simulink library "bushing_forces_lib"  (R2025a)
settings: Solver=VariableStepAuto  StartTime=0.0  StopTime=10.0  RelTol=1e-3
undefined symbols (not defined in the file): b1_radial_max, d_axial, d_axialX, d_axialY, d_axialZ, d_radial, d_tors, d_torsX, d_torsY, d_torsZ, f_axial_dam, f_axial_spr, f_axialX_dam, f_axialX_spr, f_axialY_dam, f_axialY_spr, f_axialZ_dam, f_axialZ_spr, f_radial_dam, f_radial_max, f_radial_spr, k1_radial_max, k_axial, k_axialX, k_axialY, k_axialZ, k_radial, k_tors, k_torsX, k_torsY, k_torsZ, Linear, m, m_spr, m_sprZ, m_torsY, m_torsZ, m_torX, q_spr, q_sprZ, Table, v_axial, v_axialX, v_axialY, v_axialZ, v_radial, w, w_torsY, w_torsZ, w_torX, x_axial, x_axialX, x_axialY, x_axialZ, x_radial, x_radial_max
libraries: nesl_utility x26, fl_lib x18, $bdroot x10
(part 1 of 2)
Description:
  | Copyright 2026 The MathWorks, Inc.
settings Model: Creator=smiller  LastModifiedBy=smiller
settings OptimizationCC: ReuseModelBlockBuffer=off
settings ModelReferenceCC: EnableRefExpFcnMdlSchedulingChecks=on
settings RTWCC: GPUComputeCapability=3.5

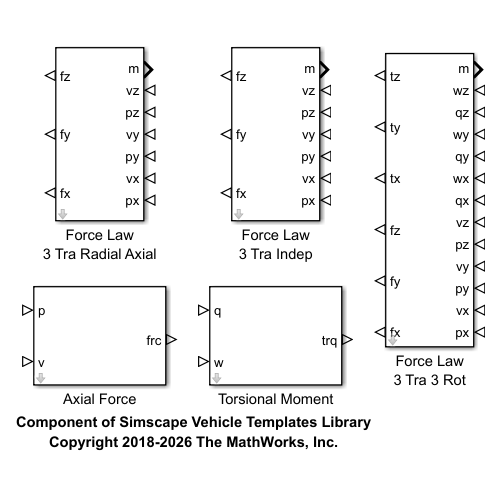
[thumbnail: Simulink's stored preview of the top-level diagram]
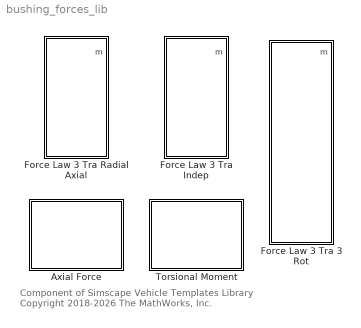
== system bushing_forces_lib ==
  note: Component of Simscape Vehicle Templates Library
      | Copyright 2018-2026 The MathWorks, Inc.
  Axial Force : Subsystem  mask(Axial Compliance){popup_force_law_spr=Linear, k_axial=k_axial, x_axial=x_axial, f_axial_spr=f_axial_spr, popup_force_law_dam=Linear, d_axial=d_axial, v_axial=v_axial, f_axial_dam=f_axial_dam}
      mask prompts: popup_force_law_spr "Spring Force Law"; k_axial "Spring Coefficient (N/mm)"; x_axial "Spring Displacement [min max] (mm)"; f_axial_spr "Spring Force [min max] (N)"; popup_force_law_dam "Damper Force Law"; d_axial "Damper Coefficient (N/(m/s))"; v_axial "Damper Velocity [min max] (m/s)"; f_axial_dam "Damper Force [min max] (N)"
      mask help: Models axial compliance of the bushing. Select force laws that model compliance as linear or nonlinear.
      mask TypeOptions popup_force_law_spr: Force Law Spring/popup_force_law
      mask Callback popup_force_law_spr:
      | maskObj = Simulink.Mask.get(gcb); % Get the mask object of the current block
      | kaxi_h  = maskObj.getParameter('k_axial'); % Get the parameter to hide
      | 
      | xaxi_h  = maskObj.getParameter('x_axial'); % Get the parameter to hide
      | fSaxi_h  = maskObj.getParameter('f_axial_spr'); % Get the parameter to hide
      | 
      | % Check the value of ControlParam
      | controlParamValue = get_param(gcb, 'popup_force_law_spr');
      | 
      | kaxi_h.Visible  = 'off';
      | xaxi_h.Visible  = 'off';
      | fSaxi_h.Visible  = 'off';
      | 
      | if strcmp(controlParamValue, 'Linear')
      |     kaxi_h.Visible  = 'on';
      | else
      |     xaxi_h.Visible  = 'on';
      |     fSaxi_h.Visible  = 'on';
      | end
      mask TypeOptions k_axial: Force Law Spring/k_axial
      mask TypeOptions x_axial: Force Law Spring/x_axial
      mask TypeOptions f_axial_spr: Force Law Spring/f_axial
      mask TypeOptions popup_force_law_dam: Force Law Damping/popup_force_law
      mask Callback popup_force_law_dam:
      | maskObj = Simulink.Mask.get(gcb); % Get the mask object of the current block
      | daxi_h  = maskObj.getParameter('d_axial'); % Get the parameter to hide
      | 
      | vaxi_h  = maskObj.getParameter('v_axial'); % Get the parameter to hide
      | fDaxi_h  = maskObj.getParameter('f_axial_dam'); % Get the parameter to hide
      | 
      | % Check the value of ControlParam
      | controlParamValue = get_param(gcb, 'popup_force_law_dam');
      | 
      | daxi_h.Visible  = 'off';
      | vaxi_h.Visible  = 'off';
      | fDaxi_h.Visible  = 'off';
      | 
      | if strcmp(controlParamValue, 'Linear')
      |     daxi_h.Visible  = 'on';
      | else
      |     vaxi_h.Visible  = 'on';
      |     fDaxi_h.Visible  = 'on';
      | end
      mask TypeOptions d_axial: Force Law Damping/d_axial
      mask TypeOptions v_axial: Force Law Damping/v_axial
      mask TypeOptions f_axial_dam: Force Law Damping/f_axial
      mask DialogControl cont_radial Prompt: Radial
  Force Law 3 Tra 3 Rot : Subsystem  mask(Bushing Compliance){popup_force_law_spr_axiX=Linear, k_axialX=k_axialX, x_axialX=x_axialX, f_axialX_spr=f_axialX_spr, popup_force_law_dam_axiX=Linear, d_axialX=d_axialX, v_axialX=v_axialX, f_axialX_dam=f_axialX_dam, popup_force_law_spr_axiY=Linear, k_axialY=k_axialY, x_axialY=x_axialY, f_axialY_spr=f_axialY_spr, popup_force_law_dam_axiY=Linear, d_axialY=d_axialY, v_axialY=v_axialY, f_axialY_dam=f_axialY_dam, popup_force_law_spr_axiZ=Linear, k_axialZ=k_axialZ, x_axialZ=x_axialZ, f_axialZ_spr=f_axialZ_spr, popup_force_law_dam_axiZ=Linear, d_axialZ=d_axialZ, f_axialZ_dam=f_axialZ_dam, v_axialZ=v_axialZ, popup_force_law_spr_torX=Linear, k_torsX=k_torsX, q_sprX=q_spr, m_sprX=m_spr, popup_force_law_dam_torX=Linear, d_torsX=d_torsX, w_torsX=w_torX, m_torsX=m_torX, popup_force_law_spr_torY=Table, k_torsY=k_torsY, q_sprY=q_spr, m_sprY=m_spr, popup_force_law_dam_torY=Table, d_torsY=d_torsY, w_torsY=w_torsY, m_torsY=m_torsY, popup_force_law_spr_torZ=Linear, k_torsZ=k_torsZ, q_sprZ=q_sprZ, m_sprZ=m_sprZ, popup_force_law_dam_torZ=Linear, d_torsZ=d_torsZ, w_torsZ=w_torsZ, m_torsZ=m_torsZ}
      mask prompts: popup_force_law_spr_axiX "Spring Force Law"; k_axialX "Spring Coefficient (N/mm)"; x_axialX "Spring Displacement [min max] (mm)"; f_axialX_spr "Spring Force [min max] (N)"; popup_force_law_dam_axiX "Damper Force Law"; d_axialX "Damper Coefficient (N/(m/s))"; v_axialX "Damper Velocity [min max] (m/s)"; f_axialX_dam "Damper Force [min max] (N)"; popup_force_law_spr_axiY "Spring Force Law"; k_axialY "Spring Coefficient (N/mm)"; x_axialY "Spring Displacement [min max] (mm)"; f_axialY_spr "Spring Force [min max] (N)"; popup_force_law_dam_axiY "Damper Force Law"; d_axialY "Damper Coefficient (N/(m/s))"; v_axialY "Damper Velocity [min max] (m/s)"; f_axialY_dam "Damper Force [min max] (N)"; popup_force_law_spr_axiZ "Spring Force Law"; k_axialZ "Spring Coefficient (N/mm)"; x_axialZ "Spring Displacement [min max] (mm)"; f_axialZ_spr "Spring Force [min max] (N)"; popup_force_law_dam_axiZ "Damper Force Law"; d_axialZ "Damper Coefficient (N/(m/s))"; f_axialZ_dam "Damper Force [min max] (N)"; v_axialZ "Damper Velocity [min max] (m/s)"; popup_force_law_spr_torX "Spring Force Law"; k_torsX "Spring Coefficient  (N*m/deg)"; q_sprX "Spring Displacement [min max] (deg)"; m_sprX "Spring Torque [min max] (N*m)"; popup_force_law_dam_torX "Damper Force Law"; d_torsX "Damper Coefficient (N*m/(deg/s))"; w_torsX "Damper Velocity [min max] (deg/s)"; m_torsX "Damper Torque [min max] (N*m)"; popup_force_law_spr_torY "Spring Force Law"; k_torsY "Spring Coefficient (N*m/deg)"; q_sprY "Spring Displacement [min max] (deg)"; m_sprY "Spring Torque [min max] (N*m)"; popup_force_law_dam_torY "Damper Force Law"; d_torsY "Damper Coefficient (N*m/(deg/s))"; w_torsY "Damper Velocity [min max] (deg/s)"; m_torsY "Damper Torque [min max] (N*m)"; popup_force_law_spr_torZ "Spring Force Law"; k_torsZ "Spring Coefficient (N*m/deg)"; q_sprZ "Spring Displacement [min max] (deg)"; m_sprZ "Spring Torque [min max] (N*m)"; popup_force_law_dam_torZ "Damper Force Law"; d_torsZ "Damper Coefficient (N*m/(deg/s))"; w_torsZ "Damper Velocity [min max] (deg/s)"; m_torsZ "Damper Torque [min max] (N*m)"
      mask help: Models radial and axial compliance of the bushing. Select force laws that model compliance as linear or nonlinear.
      mask TypeOptions popup_force_law_spr_axiX: Force X/popup_force_law_spr
      mask Callback popup_force_law_spr_axiX:
      | maskObj = Simulink.Mask.get(gcb); % Get the mask object of the current block
      | kaxiX_h  = maskObj.getParameter('k_axialX'); % Get the parameter to hide
      | 
      | xaxiX_h  = maskObj.getParameter('x_axialX'); % Get the parameter to hide
      | fSaxiX_h  = maskObj.getParameter('f_axialX_spr'); % Get the parameter to hide
      | 
      | % Check the value of ControlParam
      | controlParamValue = get_param(gcb, 'popup_force_law_spr_axiX');
      | 
      | kaxiX_h.Visible  = 'off';
      | xaxiX_h.Visible  = 'off';
      | fSaxiX_h.Visible  = 'off';
      | 
      | if strcmp(controlParamValue, 'Linear')
      |     kaxiX_h.Visible  = 'on';
      | elseif strcmp(controlParamValue, 'Table')
      |     xaxiX_h.Visible  = 'on';
      |     fSaxiX_h.Visible  = 'on';
      | end
      mask TypeOptions k_axialX: Force X/k_axial
      mask TypeOptions x_axialX: Force X/x_axial
      mask TypeOptions f_axialX_spr: Force X/f_axial_spr
      mask TypeOptions popup_force_law_dam_axiX: Force X/popup_force_law_dam
      mask Callback popup_force_law_dam_axiX:
      | maskObj = Simulink.Mask.get(gcb); % Get the mask object of the current block
      | daxiX_h  = maskObj.getParameter('d_axialX'); % Get the parameter to hide
      | 
      | vaxiX_h  = maskObj.getParameter('v_axialX'); % Get the parameter to hide
      | fDaxiX_h  = maskObj.getParameter('f_axialX_dam'); % Get the parameter to hide
      | 
      | % Check the value of ControlParam
      | controlParamValue = get_param(gcb, 'popup_force_law_dam_axiX');
      | 
      | daxiX_h.Visible  = 'off';
      | vaxiX_h.Visible  = 'off';
      | fDaxiX_h.Visible  = 'off';
      | 
      | if strcmp(controlParamValue, 'Linear')
      |     daxiX_h.Visible  = 'on';
      | else
      |     vaxiX_h.Visible  = 'on';
      |     fDaxiX_h.Visible  = 'on';
      | end
      mask TypeOptions d_axialX: Force X/d_axial
      mask TypeOptions v_axialX: Force X/v_axial
      mask TypeOptions f_axialX_dam: Force X/f_axial_dam
      mask TypeOptions popup_force_law_spr_axiY: Force Y/popup_force_law_spr
      mask Callback popup_force_law_spr_axiY:
      | maskObj = Simulink.Mask.get(gcb); % Get the mask object of the current block
      | kaxiY_h  = maskObj.getParameter('k_axialY'); % Get the parameter to hide
      | 
      | xaxiY_h  = maskObj.getParameter('x_axialY'); % Get the parameter to hide
      | fSaxiY_h  = maskObj.getParameter('f_axialY_spr'); % Get the parameter to hide
      | 
      | % Check the value of ControlParam
      | controlParamValue = get_param(gcb, 'popup_force_law_spr_axiY');
      | 
      | kaxiY_h.Visible  = 'off';
      | xaxiY_h.Visible  = 'off';
      | fSaxiY_h.Visible  = 'off';
      | 
      | if strcmp(controlParamValue, 'Linear')
      |     kaxiY_h.Visible  = 'on';
      | elseif strcmp(controlParamValue, 'Table')
      |     xaxiY_h.Visible  = 'on';
      |     fSaxiY_h.Visible  = 'on';
      | end
      mask TypeOptions k_axialY: Force Y/k_axial
      mask TypeOptions x_axialY: Force Y/x_axial
      mask TypeOptions f_axialY_spr: Force Y/f_axial_spr
      mask TypeOptions popup_force_law_dam_axiY: Force Y/popup_force_law_dam
      mask Callback popup_force_law_dam_axiY:
      | maskObj = Simulink.Mask.get(gcb); % Get the mask object of the current block
      | daxiY_h  = maskObj.getParameter('d_axialY'); % Get the parameter to hide
      | 
      | vaxiY_h  = maskObj.getParameter('v_axialY'); % Get the parameter to hide
      | fDaxiY_h  = maskObj.getParameter('f_axialY_dam'); % Get the parameter to hide
      | 
      | % Check the value of ControlParam
      | controlParamValue = get_param(gcb, 'popup_force_law_dam_axiY');
      | 
      | daxiY_h.Visible  = 'off';
      | vaxiY_h.Visible  = 'off';
      | fDaxiY_h.Visible  = 'off';
      | 
      | if strcmp(controlParamValue, 'Linear')
      |     daxiY_h.Visible  = 'on';
      | else
      |     vaxiY_h.Visible  = 'on';
      |     fDaxiY_h.Visible  = 'on';
      | end
      mask TypeOptions d_axialY: Force Y/d_axial
      mask TypeOptions v_axialY: Force Y/v_axial
      mask TypeOptions f_axialY_dam: Force Y/f_axial_dam
      mask TypeOptions popup_force_law_spr_axiZ: Force Z/popup_force_law_spr
      mask Callback popup_force_law_spr_axiZ:
      | maskObj = Simulink.Mask.get(gcb); % Get the mask object of the current block
      | kaxiZ_h  = maskObj.getParameter('k_axialZ'); % Get the parameter to hide
      | 
      | xaxiZ_h  = maskObj.getParameter('x_axialZ'); % Get the parameter to hide
      | fSaxiZ_h  = maskObj.getParameter('f_axialZ_spr'); % Get the parameter to hide
      | 
      | % Check the value of ControlParam
      | controlParamValue = get_param(gcb, 'popup_force_law_spr_axiZ');
      | 
      | kaxiZ_h.Visible  = 'off';
      | xaxiZ_h.Visible  = 'off';
      | fSaxiZ_h.Visible  = 'off';
      | 
      | if strcmp(controlParamValue, 'Linear')
      |     kaxiZ_h.Visible  = 'on';
      | elseif strcmp(controlParamValue, 'Table')
      |     xaxiZ_h.Visible  = 'on';
      |     fSaxiZ_h.Visible  = 'on';
      | end
      mask TypeOptions k_axialZ: Force Z/k_axial
      mask TypeOptions x_axialZ: Force Z/x_axial
      mask TypeOptions f_axialZ_spr: Force Z/f_axial_spr
      mask TypeOptions popup_force_law_dam_axiZ: Force Z/popup_force_law_dam
      mask Callback popup_force_law_dam_axiZ:
      | maskObj = Simulink.Mask.get(gcb); % Get the mask object of the current block
      | daxiZ_h  = maskObj.getParameter('d_axialZ'); % Get the parameter to hide
      | 
      | vaxiZ_h  = maskObj.getParameter('v_axialZ'); % Get the parameter to hide
      | fDaxiZ_h  = maskObj.getParameter('f_axialZ_dam'); % Get the parameter to hide
      | 
      | % Check the value of ControlParam
      | controlParamValue = get_param(gcb, 'popup_force_law_dam_axiZ');
      | 
      | daxiZ_h.Visible  = 'off';
      | vaxiZ_h.Visible  = 'off';
      | fDaxiZ_h.Visible  = 'off';
      | 
      | if strcmp(controlParamValue, 'Linear')
      |     daxiZ_h.Visible  = 'on';
      | else
      |     vaxiZ_h.Visible  = 'on';
      |     fDaxiZ_h.Visible  = 'on';
      | end
      mask TypeOptions d_axialZ: Force Z/d_axial
      mask TypeOptions f_axialZ_dam: Force Z/f_axial_dam
      mask TypeOptions v_axialZ: Force Z/v_axial
      mask TypeOptions popup_force_law_spr_torX: Torque X/popup_force_law_spr
      mask Callback popup_force_law_spr_torX:
      | maskObj = Simulink.Mask.get(gcb); % Get the mask object of the current block
      | ktorX_h  = maskObj.getParameter('k_torsX'); % Get the parameter to hide
      | 
      | qsprX_h  = maskObj.getParameter('q_sprX'); % Get the parameter to hide
      | msprX_h  = maskObj.getParameter('m_sprX'); % Get the parameter to hide
      | 
      | % Check the value of ControlParam
      | controlParamValue = get_param(gcb, 'popup_force_law_spr_torX');
      | 
      | ktorX_h.Visible  = 'off';
      | qsprX_h.Visible  = 'off';
      | msprX_h.Visible  = 'off';
      | 
      | if strcmp(controlParamValue, 'Linear')
      |     ktorX_h.Visible  = 'on';
      | elseif strcmp(controlParamValue, 'Table')
      |     qsprX_h.Visible  = 'on';
      |     msprX_h.Visible  = 'on';
      | end
      mask TypeOptions k_torsX: Torque X/k_tors
      mask TypeOptions q_sprX: Torque X/q_spr
      mask TypeOptions m_sprX: Torque X/m_spr
      mask TypeOptions popup_force_law_dam_torX: Torque X/popup_force_law_dam
      mask Callback popup_force_law_dam_torX:
      | maskObj = Simulink.Mask.get(gcb); % Get the mask object of the current block
      | dtorX_h  = maskObj.getParameter('d_torsX'); % Get the parameter to hide
      | 
      | wtorX_h  = maskObj.getParameter('w_torsX'); % Get the parameter to hide
      | mtorX_h  = maskObj.getParameter('m_torsX'); % Get the parameter to hide
      | 
      | % Check the value of ControlParam
      | controlParamValue = get_param(gcb, 'popup_force_law_dam_torX');
      | 
      | dtorX_h.Visible  = 'off';
      | wtorX_h.Visible  = 'off';
      | mtorX_h.Visible  = 'off';
      | 
      | if strcmp(controlParamValue, 'Linear')
      |     dtorX_h.Visible  = 'on';
      | else
      |     wtorX_h.Visible  = 'on';
      |     mtorX_h.Visible  = 'on';
      | end
      mask TypeOptions d_torsX: Torque X/d_tors
      mask TypeOptions w_torsX: Torque X/w
      mask TypeOptions m_torsX: Torque X/m
      mask TypeOptions popup_force_law_spr_torY: Torque Y/popup_force_law_spr
      mask Callback popup_force_law_spr_torY:
      | maskObj = Simulink.Mask.get(gcb); % Get the mask object of the current block
      | ktorY_h  = maskObj.getParameter('k_torsY'); % Get the parameter to hide
      | 
      | qsprY_h  = maskObj.getParameter('q_sprY'); % Get the parameter to hide
      | msprY_h  = maskObj.getParameter('m_sprY'); % Get the parameter to hide
      | 
      | % Check the value of ControlParam
      | controlParamValue = get_param(gcb, 'popup_force_law_spr_torY');
      | 
      | ktorY_h.Visible  = 'off';
      | qsprY_h.Visible  = 'off';
      | msprY_h.Visible  = 'off';
      | 
      | if strcmp(controlParamValue, 'Linear')
      |     ktorY_h.Visible  = 'on';
      | elseif strcmp(controlParamValue, 'Table')
      |     qsprY_h.Visible  = 'on';
      |     msprY_h.Visible  = 'on';
      | end
      mask TypeOptions k_torsY: Torque Y/k_tors
      mask TypeOptions q_sprY: Torque Y/q_spr
      mask TypeOptions m_sprY: Torque Y/m_spr
      mask TypeOptions popup_force_law_dam_torY: Torque Y/popup_force_law_dam
      mask Callback popup_force_law_dam_torY:
      | maskObj = Simulink.Mask.get(gcb); % Get the mask object of the current block
      | dtorY_h  = maskObj.getParameter('d_torsY'); % Get the parameter to hide
      | 
      | wtorY_h  = maskObj.getParameter('w_torsY'); % Get the parameter to hide
      | mtorY_h  = maskObj.getParameter('m_torsY'); % Get the parameter to hide
      | 
      | % Check the value of ControlParam
      | controlParamValue = get_param(gcb, 'popup_force_law_dam_torY');
      | 
      | dtorY_h.Visible  = 'off';
      | wtorY_h.Visible  = 'off';
      | mtorY_h.Visible  = 'off';
      | 
      | if strcmp(controlParamValue, 'Linear')
      |     dtorY_h.Visible  = 'on';
      | else
      |     wtorY_h.Visible  = 'on';
      |     mtorY_h.Visible  = 'on';
      | end
      mask TypeOptions d_torsY: Torque Y/d_tors
      mask TypeOptions w_torsY: Torque Y/w
      mask TypeOptions m_torsY: Torque Y/m
      mask TypeOptions popup_force_law_spr_torZ: Torque Z/popup_force_law_spr
      mask Callback popup_force_law_spr_torZ:
      | maskObj = Simulink.Mask.get(gcb); % Get the mask object of the current block
      | ktorZ_h  = maskObj.getParameter('k_torsZ'); % Get the parameter to hide
      | 
      | qsprZ_h  = maskObj.getParameter('q_sprZ'); % Get the parameter to hide
      | msprZ_h  = maskObj.getParameter('m_sprZ'); % Get the parameter to hide
      | 
      | % Check the value of ControlParam
      | controlParamValue = get_param(gcb, 'popup_force_law_spr_torZ');
      | 
      | ktorZ_h.Visible  = 'off';
      | qsprZ_h.Visible  = 'off';
      | msprZ_h.Visible  = 'off';
      | 
      | if strcmp(controlParamValue, 'Linear')
      |     ktorZ_h.Visible  = 'on';
      | elseif strcmp(controlParamValue, 'Table')
      |     qsprZ_h.Visible  = 'on';
      |     msprZ_h.Visible  = 'on';
      | end
      mask TypeOptions k_torsZ: Torque Z/k_tors
      mask TypeOptions q_sprZ: Torque Z/q_spr
      mask TypeOptions m_sprZ: Torque Z/m_spr
      mask TypeOptions popup_force_law_dam_torZ: Torque Z/popup_force_law_dam
      mask Callback popup_force_law_dam_torZ:
      | maskObj = Simulink.Mask.get(gcb); % Get the mask object of the current block
      | dtorZ_h  = maskObj.getParameter('d_torsZ'); % Get the parameter to hide
      | 
      | wtorZ_h  = maskObj.getParameter('w_torsZ'); % Get the parameter to hide
      | mtorZ_h  = maskObj.getParameter('m_torsZ'); % Get the parameter to hide
      | 
      | % Check the value of ControlParam
      | controlParamValue = get_param(gcb, 'popup_force_law_dam_torZ');
      | 
      | dtorZ_h.Visible  = 'off';
      | wtorZ_h.Visible  = 'off';
      | mtorZ_h.Visible  = 'off';
      | 
      | if strcmp(controlParamValue, 'Linear')
      |     dtorZ_h.Visible  = 'on';
      | else
      |     wtorZ_h.Visible  = 'on';
      |     mtorZ_h.Visible  = 'on';
      | end
      mask TypeOptions d_torsZ: Torque Z/d_tors
      mask TypeOptions w_torsZ: Torque Z/w
      mask TypeOptions m_torsZ: Torque Z/m
      mask DialogControl cont_axialX Prompt: Axial (local x)
      mask DialogControl cont_axialY Prompt: Axial (local y)
      mask DialogControl cont_axialZ Prompt: Axial (local z)
      mask DialogControl cont_torsX Prompt: Torsional (local x)
      mask DialogControl cont_torsY Prompt: Torsional (local y)
      mask DialogControl cont_torsZ Prompt: Torsional (local z)
  Force Law 3 Tra Indep : Subsystem  mask(Bushing Compliance){popup_force_law_spr_axiX=Linear, k_axialX=k_axialX, x_axialX=x_axialX, f_axialX_spr=f_axialX_spr, popup_force_law_dam_axiX=Linear, d_axialX=d_axialX, v_axialX=v_axialX, f_axialX_dam=f_axialX_dam, popup_force_law_spr_axiY=Linear, k_axialY=k_axialY, x_axialY=x_axialY, f_axialY_spr=f_axialY_spr, popup_force_law_dam_axiY=Linear, d_axialY=d_axialY, v_axialY=v_axialY, f_axialY_dam=f_axialY_dam, popup_force_law_spr_axiZ=Linear, k_axialZ=k_axialZ, x_axialZ=x_axialZ, f_axialZ_spr=f_axialZ_spr, popup_force_law_dam_axiZ=Linear, d_axialZ=d_axialZ, f_axialZ_dam=f_axialZ_dam, v_axialZ=v_axialZ}
      mask prompts: popup_force_law_spr_axiX "Spring Force Law"; k_axialX "Spring Coefficient (N/mm)"; x_axialX "Spring Displacement [min max] (mm)"; f_axialX_spr "Spring Force [min max] (N)"; popup_force_law_dam_axiX "Damper Force Law"; d_axialX "Damper Coefficient (N/(m/s))"; v_axialX "Damper Velocity [min max] (m/s)"; f_axialX_dam "Damper Force [min max] (N)"; popup_force_law_spr_axiY "Spring Force Law"; k_axialY "Spring Coefficient (N/mm)"; x_axialY "Spring Displacement [min max] (mm)"; f_axialY_spr "Spring Force [min max] (N)"; popup_force_law_dam_axiY "Damper Force Law"; d_axialY "Damper Coefficient (N/(m/s))"; v_axialY "Damper Velocity [min max] (m/s)"; f_axialY_dam "Damper Force [min max] (N)"; popup_force_law_spr_axiZ "Spring Force Law"; k_axialZ "Spring Coefficient (N/mm)"; x_axialZ "Spring Displacement [min max] (mm)"; f_axialZ_spr "Spring Force [min max] (N)"; popup_force_law_dam_axiZ "Damper Force Law"; d_axialZ "Damper Coefficient (N/(m/s))"; f_axialZ_dam "Damper Force [min max] (N)"; v_axialZ "Damper Velocity [min max] (m/s)"
      mask help: Models radial and axial compliance of the bushing. Select force laws that model compliance as linear or nonlinear.
      mask TypeOptions popup_force_law_spr_axiX: Force X/popup_force_law_spr
      mask Callback popup_force_law_spr_axiX:
      | maskObj = Simulink.Mask.get(gcb); % Get the mask object of the current block
      | kaxiX_h  = maskObj.getParameter('k_axialX'); % Get the parameter to hide
      | 
      | xaxiX_h  = maskObj.getParameter('x_axialX'); % Get the parameter to hide
      | fSaxiX_h  = maskObj.getParameter('f_axialX_spr'); % Get the parameter to hide
      | 
      | % Check the value of ControlParam
      | controlParamValue = get_param(gcb, 'popup_force_law_spr_axiX');
      | 
      | kaxiX_h.Visible  = 'off';
      | xaxiX_h.Visible  = 'off';
      | fSaxiX_h.Visible  = 'off';
      | 
      | if strcmp(controlParamValue, 'Linear')
      |     kaxiX_h.Visible  = 'on';
      | elseif strcmp(controlParamValue, 'Table')
      |     xaxiX_h.Visible  = 'on';
      |     fSaxiX_h.Visible  = 'on';
      | end
      mask TypeOptions k_axialX: Force X/k_axial
      mask TypeOptions x_axialX: Force X/x_axial
      mask TypeOptions f_axialX_spr: Force X/f_axial_spr
      mask TypeOptions popup_force_law_dam_axiX: Force X/popup_force_law_dam
      mask Callback popup_force_law_dam_axiX:
      | maskObj = Simulink.Mask.get(gcb); % Get the mask object of the current block
      | daxiX_h  = maskObj.getParameter('d_axialX'); % Get the parameter to hide
      | 
      | vaxiX_h  = maskObj.getParameter('v_axialX'); % Get the parameter to hide
      | fDaxiX_h  = maskObj.getParameter('f_axialX_dam'); % Get the parameter to hide
      | 
      | % Check the value of ControlParam
      | controlParamValue = get_param(gcb, 'popup_force_law_dam_axiX');
      | 
      | daxiX_h.Visible  = 'off';
      | vaxiX_h.Visible  = 'off';
      | fDaxiX_h.Visible  = 'off';
      | 
      | if strcmp(controlParamValue, 'Linear')
      |     daxiX_h.Visible  = 'on';
      | else
      |     vaxiX_h.Visible  = 'on';
      |     fDaxiX_h.Visible  = 'on';
      | end
      mask TypeOptions d_axialX: Force X/d_axial
      mask TypeOptions v_axialX: Force X/v_axial
      mask TypeOptions f_axialX_dam: Force X/f_axial_dam
      mask TypeOptions popup_force_law_spr_axiY: Force Y/popup_force_law_spr
      mask Callback popup_force_law_spr_axiY:
      | maskObj = Simulink.Mask.get(gcb); % Get the mask object of the current block
      | kaxiY_h  = maskObj.getParameter('k_axialY'); % Get the parameter to hide
      | 
      | xaxiY_h  = maskObj.getParameter('x_axialY'); % Get the parameter to hide
      | fSaxiY_h  = maskObj.getParameter('f_axialY_spr'); % Get the parameter to hide
      | 
      | % Check the value of ControlParam
      | controlParamValue = get_param(gcb, 'popup_force_law_spr_axiY');
      | 
      | kaxiY_h.Visible  = 'off';
      | xaxiY_h.Visible  = 'off';
      | fSaxiY_h.Visible  = 'off';
      | 
      | if strcmp(controlParamValue, 'Linear')
      |     kaxiY_h.Visible  = 'on';
      | elseif strcmp(controlParamValue, 'Table')
      |     xaxiY_h.Visible  = 'on';
      |     fSaxiY_h.Visible  = 'on';
      | end
      mask TypeOptions k_axialY: Force Y/k_axial
      mask TypeOptions x_axialY: Force Y/x_axial
      mask TypeOptions f_axialY_spr: Force Y/f_axial_spr
      mask TypeOptions popup_force_law_dam_axiY: Force Y/popup_force_law_dam
      mask Callback popup_force_law_dam_axiY:
      | maskObj = Simulink.Mask.get(gcb); % Get the mask object of the current block
      | daxiY_h  = maskObj.getParameter('d_axialY'); % Get the parameter to hide
      | 
      | vaxiY_h  = maskObj.getParameter('v_axialY'); % Get the parameter to hide
      | fDaxiY_h  = maskObj.getParameter('f_axialY_dam'); % Get the parameter to hide
      | 
      | % Check the value of ControlParam
      | controlParamValue = get_param(gcb, 'popup_force_law_dam_axiY');
      | 
      | daxiY_h.Visible  = 'off';
      | vaxiY_h.Visible  = 'off';
      | fDaxiY_h.Visible  = 'off';
      | 
      | if strcmp(controlParamValue, 'Linear')
      |     daxiY_h.Visible  = 'on';
      | else
      |     vaxiY_h.Visible  = 'on';
      |     fDaxiY_h.Visible  = 'on';
      | end
      mask TypeOptions d_axialY: Force Y/d_axial
      mask TypeOptions v_axialY: Force Y/v_axial
      mask TypeOptions f_axialY_dam: Force Y/f_axial_dam
      mask TypeOptions popup_force_law_spr_axiZ: Force Z/popup_force_law_spr
      mask Callback popup_force_law_spr_axiZ:
      | maskObj = Simulink.Mask.get(gcb); % Get the mask object of the current block
      | kaxiZ_h  = maskObj.getParameter('k_axialZ'); % Get the parameter to hide
      | 
      | xaxiZ_h  = maskObj.getParameter('x_axialZ'); % Get the parameter to hide
      | fSaxiZ_h  = maskObj.getParameter('f_axialZ_spr'); % Get the parameter to hide
      | 
      | % Check the value of ControlParam
      | controlParamValue = get_param(gcb, 'popup_force_law_spr_axiZ');
      | 
      | kaxiZ_h.Visible  = 'off';
      | xaxiZ_h.Visible  = 'off';
      | fSaxiZ_h.Visible  = 'off';
      | 
      | if strcmp(controlParamValue, 'Linear')
      |     kaxiZ_h.Visible  = 'on';
      | elseif strcmp(controlParamValue, 'Table')
      |     xaxiZ_h.Visible  = 'on';
      |     fSaxiZ_h.Visible  = 'on';
      | end
      mask TypeOptions k_axialZ: Force Z/k_axial
      mask TypeOptions x_axialZ: Force Z/x_axial
      mask TypeOptions f_axialZ_spr: Force Z/f_axial_spr
      mask TypeOptions popup_force_law_dam_axiZ: Force Z/popup_force_law_dam
      mask Callback popup_force_law_dam_axiZ:
      | maskObj = Simulink.Mask.get(gcb); % Get the mask object of the current block
      | daxiZ_h  = maskObj.getParameter('d_axialZ'); % Get the parameter to hide
      | 
      | vaxiZ_h  = maskObj.getParameter('v_axialZ'); % Get the parameter to hide
      | fDaxiZ_h  = maskObj.getParameter('f_axialZ_dam'); % Get the parameter to hide
      | 
      | % Check the value of ControlParam
      | controlParamValue = get_param(gcb, 'popup_force_law_dam_axiZ');
      | 
      | daxiZ_h.Visible  = 'off';
      | vaxiZ_h.Visible  = 'off';
      | fDaxiZ_h.Visible  = 'off';
      | 
      | if strcmp(controlParamValue, 'Linear')
      |     daxiZ_h.Visible  = 'on';
      | else
      |     vaxiZ_h.Visible  = 'on';
      |     fDaxiZ_h.Visible  = 'on';
      | end
      mask TypeOptions d_axialZ: Force Z/d_axial
      mask TypeOptions f_axialZ_dam: Force Z/f_axial_dam
      mask TypeOptions v_axialZ: Force Z/v_axial
      mask DialogControl cont_axialX Prompt: Axial (local x)
      mask DialogControl cont_axialY Prompt: Axial (local y)
      mask DialogControl cont_axialZ Prompt: Axial (local z)
  Force Law 3 Tra Radial Axial : Subsystem  mask(Bushing Compliance){popup_force_law_spr_rad=Linear, k_radial=k_radial, x_radial=x_radial, f_radial_spr=f_radial_spr, k1_radial_max=k1_radial_max, b1_radial_max=b1_radial_max, x_radial_max=x_radial_max, f_radial_max=f_radial_max, popup_force_law_dam_rad=Linear, d_radial=d_radial, v_radial=v_radial, f_radial_dam=f_radial_dam, popup_force_law_spr_axi=Linear, k_axial=k_axial, x_axial=x_axial, f_axial_spr=f_axial_spr, popup_force_law_dam_axi=Linear, d_axial=d_axial, v_axial=v_axial, f_axial_dam=f_axial_dam}
      mask prompts: popup_force_law_spr_rad "Spring Force Law"; k_radial "Spring Coefficient (N/mm)"; x_radial "Spring Deflection [min max] (mm)"; f_radial_spr "Spring Force [min max] (N)"; k1_radial_max "Maxwell k1"; b1_radial_max "Maxwell b1"; x_radial_max "Maxwell Displacement [min max] (mm)"; f_radial_max "Maxwell Force [min max] (N)"; popup_force_law_dam_rad "Damper Force Law"; d_radial "Damper Coefficient (N/(m/s))"; v_radial "Damper Velocity [min max] (m/s)"; f_radial_dam "Damper Force [min max] (N)"; popup_force_law_spr_axi "Spring Force Law"; k_axial "Spring Coefficient (N/mm)"; x_axial "Spring Displacement [min max] (mm)"; f_axial_spr "Spring Force [min max] (N)"; popup_force_law_dam_axi "Damper Force Law"; d_axial "Damper Coefficient (N/(m/s))"; v_axial "Damper Velocity [min max] (m/s)"; f_axial_dam "Damper Force [min max] (N)"
      mask help: Models radial and axial compliance of the bushing. Select force laws that model compliance as linear, nonlinear, or nonlinear with hysteresis.
      mask TypeOptions popup_force_law_spr_rad: Radial Force/popup_force_law_spr
      mask Callback popup_force_law_spr_rad:
      | maskObj = Simulink.Mask.get(gcb); % Get the mask object of the current block
      | krad_h  = maskObj.getParameter('k_radial'); % Get the parameter to hide
      | 
      | xrad_h  = maskObj.getParameter('x_radial'); % Get the parameter to hide
      | fSrad_h = maskObj.getParameter('f_radial_spr'); % Get the parameter to hide
      | k1rad_h  = maskObj.getParameter('k1_radial_max'); % Get the parameter to hide
      | b1rad_h  = maskObj.getParameter('b1_radial_max'); % Get the parameter to hide
      | xmrad_h  = maskObj.getParameter('x_radial_max'); % Get the parameter to hide
      | fmrad_h  = maskObj.getParameter('f_radial_max'); % Get the parameter to hide
      | 
      | % Check the value of ControlParam
      | controlParamValue = get_param(gcb, 'popup_force_law_spr_rad');
      | 
      | krad_h.Visible  = 'off';
      | xrad_h.Visible  = 'off';
      | fSrad_h.Visible = 'off';
      | k1rad_h.Visible  = 'off';
      | b1rad_h.Visible  = 'off';
      | xmrad_h.Visible  = 'off';
      | fmrad_h.Visible  = 'off';
      | 
      | if strcmp(controlParamValue, 'Linear')
      |     krad_h.Visible  = 'on';
      | elseif strcmp(controlParamValue, 'Table')
      |     xrad_h.Visible  = 'on';
      |     fSrad_h.Visible = 'on';
      | elseif strcmp(controlParamValue, 'Maxwell_SLS')
      |     k1rad_h.Visible  = 'on';
      |     b1rad_h.Visible = 'on';
      |     xmrad_h.Visible = 'on';
      |     fmrad_h.Visible = 'on';
      | end
      mask TypeOptions k_radial: Radial Force/k_radial
      mask TypeOptions x_radial: Radial Force/x_radial
      mask TypeOptions f_radial_spr: Radial Force/f_radial_spr
      mask TypeOptions k1_radial_max: Radial Force/k1_radial_max
      mask TypeOptions b1_radial_max: Radial Force/b1_radial_max
      mask TypeOptions x_radial_max: Radial Force/x_radial_max
      mask TypeOptions f_radial_max: Radial Force/f_radial_max
      mask TypeOptions popup_force_law_dam_rad: Radial Force/popup_force_law_dam
      mask Callback popup_force_law_dam_rad:
      | maskObj = Simulink.Mask.get(gcb); % Get the mask object of the current block
      | drad_h  = maskObj.getParameter('d_radial'); % Get the parameter to hide
      | 
      | vrad_h  = maskObj.getParameter('v_radial'); % Get the parameter to hide
      | fDrad_h = maskObj.getParameter('f_radial_dam'); % Get the parameter to hide
      | 
      | % Check the value of ControlParam
      | controlParamValue = get_param(gcb, 'popup_force_law_dam_rad');
      | 
      | drad_h.Visible  = 'off';
      | vrad_h.Visible  = 'off';
      | fDrad_h.Visible = 'off';
      | 
      | if strcmp(controlParamValue, 'Linear')
      |     drad_h.Visible  = 'on';
      | elseif strcmp(controlParamValue, 'Table')
      |     vrad_h.Visible  = 'on';
      |     fDrad_h.Visible = 'on';
      | end
      mask TypeOptions d_radial: Radial Force/d_radial
      mask TypeOptions v_radial: Radial Force/v_radial
      mask TypeOptions f_radial_dam: Radial Force/f_radial_dam
      mask TypeOptions popup_force_law_spr_axi: Axial Force/popup_force_law_spr
      mask Callback popup_force_law_spr_axi:
      | maskObj = Simulink.Mask.get(gcb); % Get the mask object of the current block
      | kaxi_h  = maskObj.getParameter('k_axial'); % Get the parameter to hide
      | 
      | xaxi_h  = maskObj.getParameter('x_axial'); % Get the parameter to hide
      | fSaxi_h  = maskObj.getParameter('f_axial_spr'); % Get the parameter to hide
      | 
      | % Check the value of ControlParam
      | controlParamValue = get_param(gcb, 'popup_force_law_spr_axi');
      | 
      | kaxi_h.Visible  = 'off';
      | xaxi_h.Visible  = 'off';
      | fSaxi_h.Visible  = 'off';
      | 
      | if strcmp(controlParamValue, 'Linear')
      |     kaxi_h.Visible  = 'on';
      | elseif strcmp(controlParamValue, 'Table')
      |     xaxi_h.Visible  = 'on';
      |     fSaxi_h.Visible  = 'on';
      | end
      mask TypeOptions k_axial: Axial Force/k_axial
      mask TypeOptions x_axial: Axial Force/x_axial
      mask TypeOptions f_axial_spr: Axial Force/f_axial_spr
      mask TypeOptions popup_force_law_dam_axi: Axial Force/popup_force_law_dam
      mask Callback popup_force_law_dam_axi:
      | maskObj = Simulink.Mask.get(gcb); % Get the mask object of the current block
      | daxi_h  = maskObj.getParameter('d_axial'); % Get the parameter to hide
      | 
      | vaxi_h  = maskObj.getParameter('v_axial'); % Get the parameter to hide
      | fDaxi_h  = maskObj.getParameter('f_axial_dam'); % Get the parameter to hide
      | 
      | % Check the value of ControlParam
      | controlParamValue = get_param(gcb, 'popup_force_law_dam_axi');
      | 
      | daxi_h.Visible  = 'off';
      | vaxi_h.Visible  = 'off';
      | fDaxi_h.Visible  = 'off';
      | 
      | if strcmp(controlParamValue, 'Linear')
      |     daxi_h.Visible  = 'on';
      | else
      |     vaxi_h.Visible  = 'on';
      |     fDaxi_h.Visible  = 'on';
      | end
      mask TypeOptions d_axial: Axial Force/d_axial
      mask TypeOptions v_axial: Axial Force/v_axial
      mask TypeOptions f_axial_dam: Axial Force/f_axial_dam
      mask DialogControl cont_radial Prompt: Radial
      mask DialogControl cont_axial Prompt: Axial
  Torsional Moment : Subsystem  mask(Axial Compliance){popup_force_law_spr=Linear, k_tors=k_tors, q_spr=q_spr, m_spr=m_spr, popup_force_law_dam=Linear, d_tors=d_tors, m=m, w=w}
      mask prompts: popup_force_law_spr "Spring Force Law"; k_tors "Spring Stiffness (N*m/deg)"; q_spr "Spring Displacement [min max] (deg)"; m_spr "Spring Torque [min max] (N*m)"; popup_force_law_dam "Damper Force Law"; d_tors "Damping Coefficient (N*m/(deg/s))"; m "Damper Torque [min max] (N*m)"; w "Damper Velocity [min max] (deg/s)"
      mask help: Models axial compliance of the bushing. Select force laws that model compliance as linear or nonlinear.
      mask TypeOptions popup_force_law_spr: Force Law Spring/popup_force_law
      mask Callback popup_force_law_spr:
      | maskObj = Simulink.Mask.get(gcb); % Get the mask object of the current block
      | ktor_h  = maskObj.getParameter('k_tors'); % Get the parameter to hide
      | 
      | qspr_h  = maskObj.getParameter('q_spr'); % Get the parameter to hide
      | mspr_h  = maskObj.getParameter('m_spr'); % Get the parameter to hide
      | 
      | % Check the value of ControlParam
      | controlParamValue = get_param(gcb, 'popup_force_law_spr');
      | 
      | ktor_h.Visible  = 'off';
      | qspr_h.Visible  = 'off';
      | mspr_h.Visible  = 'off';
      | 
      | if strcmp(controlParamValue, 'Linear')
      |     ktor_h.Visible  = 'on';
      | else
      |     qspr_h.Visible  = 'on';
      |     mspr_h.Visible  = 'on';
      | end
      mask TypeOptions k_tors: Force Law Spring/k_tors
      mask TypeOptions q_spr: Force Law Spring/q
      mask TypeOptions m_spr: Force Law Spring/m
      mask TypeOptions popup_force_law_dam: Force Law Damping/popup_force_law
      mask Callback popup_force_law_dam:
      | maskObj = Simulink.Mask.get(gcb); % Get the mask object of the current block
      | dtor_h  = maskObj.getParameter('d_tors'); % Get the parameter to hide
      | 
      | w_h  = maskObj.getParameter('w'); % Get the parameter to hide
      | m_h  = maskObj.getParameter('m'); % Get the parameter to hide
      | 
      | % Check the value of ControlParam
      | controlParamValue = get_param(gcb, 'popup_force_law_dam');
      | 
      | dtor_h.Visible  = 'off';
      | w_h.Visible  = 'off';
      | m_h.Visible  = 'off';
      | 
      | if strcmp(controlParamValue, 'Linear')
      |     dtor_h.Visible  = 'on';
      | else
      |     w_h.Visible  = 'on';
      |     m_h.Visible  = 'on';
      | end
      mask TypeOptions d_tors: Force Law Damping/d_tors
      mask TypeOptions m: Force Law Damping/m
      mask TypeOptions w: Force Law Damping/w
      mask DialogControl cont_radial Prompt: Radial

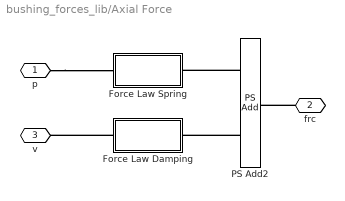
== system bushing_forces_lib/Axial Force ==
  Force Law Damping : Subsystem  Variant=on  VariantControlMode=label  VariantControl=Choice  LabelModeActiveChoice=Linear  mask(Compliance Damping){popup_force_law=Linear, d_axial=d_axial, v_axial=v_axial, f_axial=f_axial_dam}
      mask prompts: popup_force_law "Force Law"; d_axial "Linear Damping (N/(m/s))"; v_axial "Table Velocity (m/s)"; f_axial "Table Force (N)"
      mask help: Models damping of the compliance element using linear or nonlinear models.
      mask init:
      | if(strcmp(get_param(gcb, 'popup_force_law'),'Linear'))
      |     set_param(gcb,'LabelModeActiveChoice','Linear')
      | else
      |     set_param(gcb,'LabelModeActiveChoice','Table')
      | end
      mask TypeOptions popup_force_law: Linear | Table
      mask Callback popup_force_law:
      | maskObj = Simulink.Mask.get(gcb); % Get the mask object of the current block
      | daxi_h  = maskObj.getParameter('d_axial'); % Get the parameter to hide
      | 
      | vaxi_h  = maskObj.getParameter('v_axial'); % Get the parameter to hide
      | faxi_h = maskObj.getParameter('f_axial'); % Get the parameter to hide
      | 
      | % Check the value of ControlParam
      | controlParamValue = get_param(gcb, 'popup_force_law');
      | 
      | daxi_h.Visible  = 'off';
      | vaxi_h.Visible  = 'off';
      | faxi_h.Visible = 'off';
      | 
      | if strcmp(controlParamValue, 'Linear')
      |     daxi_h.Visible  = 'on';
      | else
      |     vaxi_h.Visible  = 'on';
      |     faxi_h.Visible = 'on';
      | end
  Force Law Spring : Subsystem  Variant=on  VariantControlMode=label  VariantControl=Choice  LabelModeActiveChoice=Linear  mask(Compliance Stiffness){popup_force_law=Linear, k_axial=k_axial, x_axial=x_axial, f_axial=f_axial_spr}
      mask prompts: popup_force_law "Force Law"; k_axial "Linear Stiffness (N/mm)"; x_axial "Table Displacement (mm)"; f_axial "Table Force (N)"
      mask help: Models stiffness of the compliance element using linear or nonlinear models.
      mask init:
      | if(strcmp(get_param(gcb, 'popup_force_law'),'Linear'))
      |     set_param(gcb,'LabelModeActiveChoice','Linear')
      | else
      |     set_param(gcb,'LabelModeActiveChoice','Table')
      | end
      mask TypeOptions popup_force_law: Linear | Table
      mask Callback popup_force_law:
      | maskObj = Simulink.Mask.get(gcb); % Get the mask object of the current block
      | kaxi_h  = maskObj.getParameter('k_axial'); % Get the parameter to hide
      | 
      | xaxi_h  = maskObj.getParameter('x_axial'); % Get the parameter to hide
      | faxi_h  = maskObj.getParameter('f_axial'); % Get the parameter to hide
      | 
      | % Check the value of ControlParam
      | controlParamValue = get_param(gcb, 'popup_force_law');
      | 
      | kaxi_h.Visible  = 'off';
      | xaxi_h.Visible  = 'off';
      | faxi_h.Visible  = 'off';
      | 
      | if strcmp(controlParamValue, 'Linear')
      |     kaxi_h.Visible  = 'on';
      | else
      |     xaxi_h.Visible  = 'on';
      |     faxi_h.Visible  = 'on';
      | end
  PS Add2 : fl_lib/Physical Signals/Functions/PS Add
  p : PMIOPort  Side=Left
  frc : PMIOPort  Port=2  Side=Right
  v : PMIOPort  Port=3  Side=Left
  connections:
  frc/RConn1 -- PS Add2/RConn1
  PS Add2/LConn2 -- Force Law Damping/RConn1
  Force Law Damping/LConn1 -- v/RConn1
  p/RConn1 -- Force Law Spring/LConn1
  PS Add2/LConn1 -- Force Law Spring/RConn1

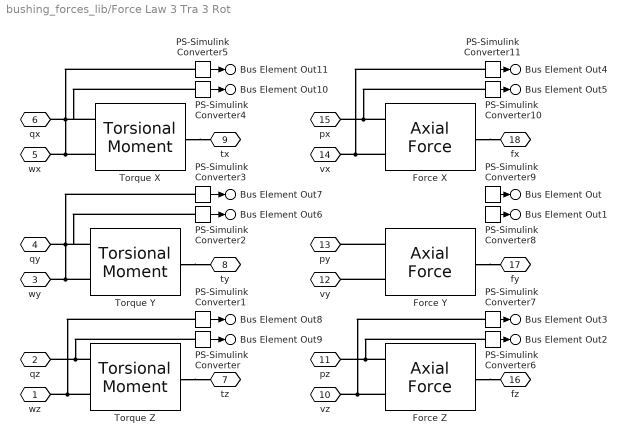
== system bushing_forces_lib/Force Law 3 Tra 3 Rot ==
  Force X : $bdroot/Axial Force  popup_force_law_spr=Linear  k_axial=k_axialX  x_axial=x_axialX  f_axial_spr=f_axialX_spr  popup_force_law_dam=Linear  d_axial=d_axialX  v_axial=v_axialX  f_axial_dam=f_axialX_dam
  Force Y : $bdroot/Axial Force  popup_force_law_spr=Linear  k_axial=k_axialY  x_axial=x_axialY  f_axial_spr=f_axialY_spr  popup_force_law_dam=Linear  d_axial=d_axialY  v_axial=v_axialY  f_axial_dam=f_axialY_dam
  Force Z : $bdroot/Axial Force  popup_force_law_spr=Linear  k_axial=k_axialZ  x_axial=x_axialZ  f_axial_spr=f_axialZ_spr  popup_force_law_dam=Linear  d_axial=d_axialZ  v_axial=v_axialZ  f_axial_dam=f_axialZ_dam
  PS-Simulink Converter : nesl_utility/PS-Simulink Converter  PhysicalDomain=network_engine_domain  SubClassName=ps_output  LeftPortType=input  RightPortType=output  PseudoPeriodic=off  Frequencies=[]  VectorFormat=inherit  Unit=deg  AffineConversion=off
  PS-Simulink Converter1 : nesl_utility/PS-Simulink Converter  PhysicalDomain=network_engine_domain  SubClassName=ps_output  LeftPortType=input  RightPortType=output  PseudoPeriodic=off  Frequencies=[]  VectorFormat=inherit  Unit=deg/s  AffineConversion=off
  PS-Simulink Converter10 : nesl_utility/PS-Simulink Converter  PhysicalDomain=network_engine_domain  SubClassName=ps_output  LeftPortType=input  RightPortType=output  PseudoPeriodic=off  Frequencies=[]  VectorFormat=inherit  Unit=mm  AffineConversion=off
  PS-Simulink Converter11 : nesl_utility/PS-Simulink Converter  PhysicalDomain=network_engine_domain  SubClassName=ps_output  LeftPortType=input  RightPortType=output  PseudoPeriodic=off  Frequencies=[]  VectorFormat=inherit  Unit=m/s  AffineConversion=off
  PS-Simulink Converter2 : nesl_utility/PS-Simulink Converter  PhysicalDomain=network_engine_domain  SubClassName=ps_output  LeftPortType=input  RightPortType=output  PseudoPeriodic=off  Frequencies=[]  VectorFormat=inherit  Unit=deg  AffineConversion=off
  PS-Simulink Converter3 : nesl_utility/PS-Simulink Converter  PhysicalDomain=network_engine_domain  SubClassName=ps_output  LeftPortType=input  RightPortType=output  PseudoPeriodic=off  Frequencies=[]  VectorFormat=inherit  Unit=deg/s  AffineConversion=off
  PS-Simulink Converter4 : nesl_utility/PS-Simulink Converter  PhysicalDomain=network_engine_domain  SubClassName=ps_output  LeftPortType=input  RightPortType=output  PseudoPeriodic=off  Frequencies=[]  VectorFormat=inherit  Unit=deg  AffineConversion=off
  PS-Simulink Converter5 : nesl_utility/PS-Simulink Converter  PhysicalDomain=network_engine_domain  SubClassName=ps_output  LeftPortType=input  RightPortType=output  PseudoPeriodic=off  Frequencies=[]  VectorFormat=inherit  Unit=deg/s  AffineConversion=off
  PS-Simulink Converter6 : nesl_utility/PS-Simulink Converter  PhysicalDomain=network_engine_domain  SubClassName=ps_output  LeftPortType=input  RightPortType=output  PseudoPeriodic=off  Frequencies=[]  VectorFormat=inherit  Unit=mm  AffineConversion=off
  PS-Simulink Converter7 : nesl_utility/PS-Simulink Converter  PhysicalDomain=network_engine_domain  SubClassName=ps_output  LeftPortType=input  RightPortType=output  PseudoPeriodic=off  Frequencies=[]  VectorFormat=inherit  Unit=m/s  AffineConversion=off
  PS-Simulink Converter8 : nesl_utility/PS-Simulink Converter  PhysicalDomain=network_engine_domain  SubClassName=ps_output  LeftPortType=input  RightPortType=output  PseudoPeriodic=off  Frequencies=[]  VectorFormat=inherit  Unit=mm  AffineConversion=off
  PS-Simulink Converter9 : nesl_utility/PS-Simulink Converter  PhysicalDomain=network_engine_domain  SubClassName=ps_output  LeftPortType=input  RightPortType=output  PseudoPeriodic=off  Frequencies=[]  VectorFormat=inherit  Unit=m/s  AffineConversion=off
  Torque X : $bdroot/Torsional Moment  popup_force_law_spr=Linear  k_tors=k_torsX  q_spr=q_sprX  m_spr=m_sprX  popup_force_law_dam=Linear  d_tors=d_torsX  m=m_torsX  w=w_torsX
  Torque Y : $bdroot/Torsional Moment  popup_force_law_spr=Table  k_tors=k_torsY  q_spr=q_sprY  m_spr=m_sprY  popup_force_law_dam=Table  d_tors=d_torsY  m=m_torsY  w=w_torsY
  Torque Z : $bdroot/Torsional Moment  popup_force_law_spr=Linear  k_tors=k_torsZ  q_spr=q_sprZ  m_spr=m_sprZ  popup_force_law_dam=Linear  d_tors=d_torsZ  m=m_torsZ  w=w_torsZ
  wz : PMIOPort  Side=Right
  qz : PMIOPort  Port=2  Side=Right
  wy : PMIOPort  Port=3  Side=Right
  qy : PMIOPort  Port=4  Side=Right
  wx : PMIOPort  Port=5  Side=Right
  qx : PMIOPort  Port=6  Side=Right
  tz : PMIOPort  Port=7  Side=Left
  ty : PMIOPort  Port=8  Side=Left
  tx : PMIOPort  Port=9  Side=Left
  vz : PMIOPort  Port=10  Side=Right
  pz : PMIOPort  Port=11  Side=Right
  vy : PMIOPort  Port=12  Side=Right
  py : PMIOPort  Port=13  Side=Right
  vx : PMIOPort  Port=14  Side=Right
  px : PMIOPort  Port=15  Side=Right
  fz : PMIOPort  Port=16  Side=Left
  fy : PMIOPort  Port=17  Side=Left
  fx : PMIOPort  Port=18  Side=Left
  Bus Element Out : Outport  PortName=m  Element=vy
  Bus Element Out1 : Outport  PortName=m  Element=py
  Bus Element Out2 : Outport  PortName=m  Element=pz
  Bus Element Out3 : Outport  PortName=m  Element=vz
  Bus Element Out4 : Outport  PortName=m  Element=vx
  Bus Element Out5 : Outport  PortName=m  Element=px
  Bus Element Out6 : Outport  PortName=m  Element=qy
  Bus Element Out7 : Outport  PortName=m  Element=wy
  Bus Element Out8 : Outport  PortName=m  Element=wz
  Bus Element Out9 : Outport  PortName=m  Element=qz
  Bus Element Out10 : Outport  PortName=m  Element=qx
  Bus Element Out11 : Outport  PortName=m  Element=wx
  wires:
  PS-Simulink Converter5/1 -> Bus Element Out11/1
  PS-Simulink Converter4/1 -> Bus Element Out10/1
  PS-Simulink Converter2/1 -> Bus Element Out6/1
  PS-Simulink Converter3/1 -> Bus Element Out7/1
  PS-Simulink Converter/1 -> Bus Element Out9/1
  PS-Simulink Converter1/1 -> Bus Element Out8/1
  PS-Simulink Converter7/1 -> Bus Element Out3/1
  PS-Simulink Converter6/1 -> Bus Element Out2/1
  PS-Simulink Converter9/1 -> Bus Element Out/1
  PS-Simulink Converter8/1 -> Bus Element Out1/1
  PS-Simulink Converter10/1 -> Bus Element Out5/1
  PS-Simulink Converter11/1 -> Bus Element Out4/1
  connections:
  wy/RConn1 -- Torque Y/LConn2 -- PS-Simulink Converter3/LConn1
  wx/RConn1 -- Torque X/LConn2 -- PS-Simulink Converter5/LConn1
  qx/RConn1 -- Torque X/LConn1 -- PS-Simulink Converter4/LConn1
  qy/RConn1 -- Torque Y/LConn1 -- PS-Simulink Converter2/LConn1
  Torque X/RConn1 -- tx/RConn1
  Torque Y/RConn1 -- ty/RConn1
  PS-Simulink Converter/LConn1 -- Torque Z/LConn1 -- qz/RConn1
  Torque Z/RConn1 -- tz/RConn1
  PS-Simulink Converter1/LConn1 -- Torque Z/LConn2 -- wz/RConn1
  vx/RConn1 -- Force X/LConn2 -- PS-Simulink Converter11/LConn1
  PS-Simulink Converter10/LConn1 -- px/RConn1 -- Force X/LConn1
  PS-Simulink Converter6/LConn1 -- pz/RConn1 -- Force Z/LConn1
  PS-Simulink Converter7/LConn1 -- Force Z/LConn2 -- vz/RConn1
  Force X/RConn1 -- fx/RConn1
  Force Y/RConn1 -- fy/RConn1
  Force Z/RConn1 -- fz/RConn1
  Force Y/LConn1 -- py/RConn1
  Force Y/LConn2 -- vy/RConn1
